simulink model "ECU1119_18b_st"  (R2018b)
settings: Solver=FixedStepDiscrete  StartTime=0.0  StopTime=10.0  RelTol=1e-3
InitFcn:
  | mbd_mpc_consistency_checks(bdroot(gcs));
values from neighbouring files (symbols this model uses):
  ANRtarget = 1.05    [Engine_init.m]
  EGRKi = 0.03    [Engine_init.m]
  EGRKp = 1.2*3    (= 3.6)    [Engine_init.m]
  EGRMax = 1    [Engine_init.m]
  EGRMin = 0    [Engine_init.m]
  EGRTgt = [0.25,0.22,0.20,0.18,0.16,0.12,0.10 ... (first row only)    [Engine_init.m]
  EGRTgt_x = [700,1200,1400,1600,1800,2000,2200]    [Engine_init.m]
  EGRTgt_y = [20,60,100,140,160]    [Engine_init.m]
  EngineSpdTgt = [700:150:2200]    [Engine_init.m]
  EngineSpdTgt_x = [0:10:100]    [Engine_init.m]
  FuelCyleMax = [40,50,60,60,60 ... (first row only)    [Engine_init.m]
  FuelCyleMax_x = [120,180,240,300,360]    [Engine_init.m]
  FuelCyleMax_y = [700,1200,1400,1600,1800,2000,2200]    [Engine_init.m]
  FuelCyleMaxSw = 0    [Engine_init.m]
  FuelCyleMin = 10    [Engine_init.m]
  FuelKd = 0    [Engine_init.m]
  FuelKi = 0.009*5    (= 0.045)    [Engine_init.m]
  FuelKp = 0.03*5    (= 0.15)    [Engine_init.m]
  Regen_Enable_SW = true    [Engine_init.m]
  Soot_Load_Off = 4    [Engine_init.m]
  Soot_Load_On = 18    [Engine_init.m]
  T_regen_max = 680    [Engine_init.m]
  T_regen_min = 550    [Engine_init.m]
undefined symbols (not defined in the file or in its folder): fifo_0_vect, fifo_1_vect, LQFP, pts1_fifo_0_vect, pts1_fifo_1_vect, pts2_fifo_0_vect, pts2_fifo_1_vect, pts3_fifo_0_vect, pts3_fifo_1_vect, pts4_fifo_0_vect, pts4_fifo_1_vect
libraries: mbd_mpc574x_ec_toolbox x111, simulink x12, canmsglib x8
(part 4 of 5)

== system ECU1119_18b_st/SigIn/PWM/PWM_PTS2 ==
  Add : Sum  Inputs=+-  AccumDataTypeStr=single
  Add1 : Sum  Inputs=+-  AccumDataTypeStr=single
  Data Store Memory : DataStoreMemory  DataStoreName=pts2_pwm_cnt  ReadBeforeWriteMsg=warning  WriteAfterWriteMsg=warning  WriteAfterReadMsg=warning  ShowAdditionalParam=off  OutDataTypeStr=uint8
  Data Store Memory2 : DataStoreMemory  DataStoreName=pts2_fifo_1_vect  ReadBeforeWriteMsg=warning  WriteAfterWriteMsg=warning  WriteAfterReadMsg=warning  InitialValue=[0 0 0 0 0 0 0 0]  ShowAdditionalParam=off  OutDataTypeStr=uint16
  Data Store Memory4 : DataStoreMemory  DataStoreName=pts2_fifo_0_vect  ReadBeforeWriteMsg=warning  WriteAfterWriteMsg=warning  WriteAfterReadMsg=warning  InitialValue=[0 0 0 0 0 0 0 0]  ShowAdditionalParam=off  OutDataTypeStr=uint16
  Data Store Read : DataStoreRead  DataStoreName=pts2_fifo_0_vect  DataStoreElements=pts2_fifo_0_vect(2)#pts2_fifo_0_vect(1)
  Data Store Read1 : DataStoreRead  DataStoreName=pts2_fifo_1_vect  DataStoreElements=pts2_fifo_1_vect(1)
  Data Store Read2 : DataStoreRead  DataStoreName=pts2_fifo_0_vect  DataStoreElements=pts2_fifo_0_vect(1)
  Data Store Write3 : DataStoreWrite  DataStoreName=pts2_fifo_0_vect
  Data Store Write5 : DataStoreWrite  DataStoreName=pts2_fifo_1_vect
  Divide : Product  Inputs=*/  OutDataTypeStr=single
  Divide1 : Product  Inputs=*//
  Freq_MC : Constant  Value=80000000  OutDataTypeStr=single
  Prescaler : Constant  Value=32  OutDataTypeStr=single
  Subsystem : Subsystem
  Subsystem_capture : Subsystem
  Terminator1 : Terminator
  Terminator2 : Terminator
  eTimer_ISR : mbd_mpc574x_ec_toolbox/Motor Control Blocks/eTIMER Blocks/eTimer_ISR_Handler  etimerModule=1  etimerInterrupt=Channel Interrupt  etimerChannel=3  etimerIsrPriority=14
      settings: SourceProductName=NXP Model-Based Design Toolbox for MPC57xx MCUs
  DC : Outport
  freq : Outport  Port=2
  wires:
  Subsystem/1(Out1) -> DC/1
  Divide/1 -> Subsystem/1(In1)
  Data Store Read/1 -> Add/1
  Divide1/1 -> freq/1
  Data Store Read2/1 -> Add1/2
  Add1/1 -> Divide/1
  Freq_MC/1 -> Divide1/1
  Data Store Read/2 -> Add/2
  Data Store Read1/1 -> Add1/1
  Add/1 -> Divide1/3, Divide/2
  Prescaler/1 -> Divide1/2
  eTimer_ISR/1 -> Subsystem_capture/Trigger
  Subsystem_capture/2(Out2) -> Data Store Write3/1
  Subsystem_capture/4(Out4) -> Data Store Write5/1
  Subsystem_capture/3(Out3) -> Terminator2/1
  Subsystem_capture/1(Out1) -> Terminator1/1
  eTimer_ISR/2 -> Subsystem_capture/1(In1)

== system ECU1119_18b_st/SigIn/PWM/PWM_PTS3 ==
  Add : Sum  Inputs=+-  AccumDataTypeStr=single
  Add1 : Sum  Inputs=+-  AccumDataTypeStr=single
  Data Store Memory : DataStoreMemory  DataStoreName=pts3_pwm_cnt  ReadBeforeWriteMsg=warning  WriteAfterWriteMsg=warning  WriteAfterReadMsg=warning  ShowAdditionalParam=off  OutDataTypeStr=uint8
  Data Store Memory2 : DataStoreMemory  DataStoreName=pts3_fifo_1_vect  ReadBeforeWriteMsg=warning  WriteAfterWriteMsg=warning  WriteAfterReadMsg=warning  InitialValue=[0 0 0 0 0 0 0 0]  ShowAdditionalParam=off  OutDataTypeStr=uint16
  Data Store Memory4 : DataStoreMemory  DataStoreName=pts3_fifo_0_vect  ReadBeforeWriteMsg=warning  WriteAfterWriteMsg=warning  WriteAfterReadMsg=warning  InitialValue=[0 0 0 0 0 0 0 0]  ShowAdditionalParam=off  OutDataTypeStr=uint16
  Data Store Read : DataStoreRead  DataStoreName=pts3_fifo_0_vect  DataStoreElements=pts3_fifo_0_vect(2)#pts3_fifo_0_vect(1)
  Data Store Read1 : DataStoreRead  DataStoreName=pts3_fifo_1_vect  DataStoreElements=pts3_fifo_1_vect(1)
  Data Store Read2 : DataStoreRead  DataStoreName=pts3_fifo_0_vect  DataStoreElements=pts3_fifo_0_vect(1)
  Data Store Write3 : DataStoreWrite  DataStoreName=pts3_fifo_0_vect
  Data Store Write5 : DataStoreWrite  DataStoreName=pts3_fifo_1_vect
  Divide : Product  Inputs=*/  OutDataTypeStr=single
  Divide1 : Product  Inputs=*//
  Freq_MC : Constant  Value=80000000  OutDataTypeStr=single
  Prescaler : Constant  Value=32  OutDataTypeStr=single
  Subsystem : Subsystem
  Subsystem_capture : Subsystem
  Terminator1 : Terminator
  Terminator2 : Terminator
  eTimer_ISR : mbd_mpc574x_ec_toolbox/Motor Control Blocks/eTIMER Blocks/eTimer_ISR_Handler  etimerModule=1  etimerInterrupt=Channel Interrupt  etimerChannel=1  etimerIsrPriority=14
      settings: SourceProductName=NXP Model-Based Design Toolbox for MPC57xx MCUs
  DC : Outport
  freq : Outport  Port=2
  wires:
  eTimer_ISR/2 -> Subsystem_capture/1(In1)
  Subsystem_capture/1(Out1) -> Terminator1/1
  Subsystem_capture/3(Out3) -> Terminator2/1
  Subsystem_capture/4(Out4) -> Data Store Write5/1
  Subsystem_capture/2(Out2) -> Data Store Write3/1
  eTimer_ISR/1 -> Subsystem_capture/Trigger
  Prescaler/1 -> Divide1/2
  Add/1 -> Divide/2, Divide1/3
  Data Store Read1/1 -> Add1/1
  Data Store Read/2 -> Add/2
  Freq_MC/1 -> Divide1/1
  Add1/1 -> Divide/1
  Data Store Read2/1 -> Add1/2
  Divide1/1 -> freq/1
  Data Store Read/1 -> Add/1
  Divide/1 -> Subsystem/1(In1)
  Subsystem/1(Out1) -> DC/1

== system ECU1119_18b_st/SigIn/PWM/PWM_PTS4 ==
  Add : Sum  Inputs=+-  AccumDataTypeStr=single
  Add1 : Sum  Inputs=+-  AccumDataTypeStr=single
  Data Store Memory : DataStoreMemory  DataStoreName=pts4_pwm_cnt  ReadBeforeWriteMsg=warning  WriteAfterWriteMsg=warning  WriteAfterReadMsg=warning  ShowAdditionalParam=off  OutDataTypeStr=uint8
  Data Store Memory2 : DataStoreMemory  DataStoreName=pts4_fifo_1_vect  ReadBeforeWriteMsg=warning  WriteAfterWriteMsg=warning  WriteAfterReadMsg=warning  InitialValue=[0 0 0 0 0 0 0 0]  ShowAdditionalParam=off  OutDataTypeStr=uint16
  Data Store Memory4 : DataStoreMemory  DataStoreName=pts4_fifo_0_vect  ReadBeforeWriteMsg=warning  WriteAfterWriteMsg=warning  WriteAfterReadMsg=warning  InitialValue=[0 0 0 0 0 0 0 0]  ShowAdditionalParam=off  OutDataTypeStr=uint16
  Data Store Read : DataStoreRead  DataStoreName=pts4_fifo_0_vect  DataStoreElements=pts4_fifo_0_vect(2)#pts4_fifo_0_vect(1)
  Data Store Read1 : DataStoreRead  DataStoreName=pts4_fifo_1_vect  DataStoreElements=pts4_fifo_1_vect(1)
  Data Store Read2 : DataStoreRead  DataStoreName=pts4_fifo_0_vect  DataStoreElements=pts4_fifo_0_vect(1)
  Data Store Write3 : DataStoreWrite  DataStoreName=pts4_fifo_0_vect
  Data Store Write5 : DataStoreWrite  DataStoreName=pts4_fifo_1_vect
  Divide : Product  Inputs=*/  OutDataTypeStr=single
  Divide1 : Product  Inputs=*//
  Freq_MC : Constant  Value=80000000  OutDataTypeStr=single
  Prescaler : Constant  Value=32  OutDataTypeStr=single
  Subsystem : Subsystem
  Subsystem_capture : Subsystem
  Terminator1 : Terminator
  Terminator2 : Terminator
  eTimer_ISR : mbd_mpc574x_ec_toolbox/Motor Control Blocks/eTIMER Blocks/eTimer_ISR_Handler  etimerModule=0  etimerInterrupt=Channel Interrupt  etimerChannel=2  etimerIsrPriority=14
      settings: SourceProductName=NXP Model-Based Design Toolbox for MPC57xx MCUs
  DC : Outport
  freq : Outport  Port=2
  wires:
  Subsystem/1(Out1) -> DC/1
  Divide/1 -> Subsystem/1(In1)
  Data Store Read/1 -> Add/1
  Divide1/1 -> freq/1
  Data Store Read2/1 -> Add1/2
  Add1/1 -> Divide/1
  Freq_MC/1 -> Divide1/1
  Data Store Read/2 -> Add/2
  Data Store Read1/1 -> Add1/1
  Add/1 -> Divide1/3, Divide/2
  Prescaler/1 -> Divide1/2
  eTimer_ISR/1 -> Subsystem_capture/Trigger
  Subsystem_capture/2(Out2) -> Data Store Write3/1
  Subsystem_capture/4(Out4) -> Data Store Write5/1
  Subsystem_capture/3(Out3) -> Terminator2/1
  Subsystem_capture/1(Out1) -> Terminator1/1
  eTimer_ISR/2 -> Subsystem_capture/1(In1)

== system ECU1119_18b_st/SigIn/PWM/Subsystem ==
  Data Store Memory1 : DataStoreMemory  DataStoreName=fifo_1_value  ReadBeforeWriteMsg=warning  WriteAfterWriteMsg=warning  WriteAfterReadMsg=warning  VectorParams1D=off  ShowAdditionalParam=off  OutDataTypeStr=uint16
  Data Store Memory3 : DataStoreMemory  DataStoreName=fifo_0_value  ReadBeforeWriteMsg=warning  WriteAfterWriteMsg=warning  WriteAfterReadMsg=warning  VectorParams1D=off  ShowAdditionalParam=off  OutDataTypeStr=uint16
  Data Store Memory5 : DataStoreMemory  DataStoreName=frequency  ReadBeforeWriteMsg=warning  WriteAfterWriteMsg=warning  WriteAfterReadMsg=warning  VectorParams1D=off  ShowAdditionalParam=off  OutDataTypeStr=single
  Data Store Memory6 : DataStoreMemory  DataStoreName=duty_cycle  ReadBeforeWriteMsg=warning  WriteAfterWriteMsg=warning  WriteAfterReadMsg=warning  VectorParams1D=off  ShowAdditionalParam=off  OutDataTypeStr=single
  Data Store Write10 : DataStoreWrite  DataStoreName=fifo_0_vect
  Data Store Write11 : DataStoreWrite  DataStoreName=fifo_1_value
  Data Store Write12 : DataStoreWrite  DataStoreName=fifo_1_vect
  Data Store Write13 : DataStoreWrite  DataStoreName=duty_cycle
  Data Store Write8 : DataStoreWrite  DataStoreName=frequency
  Data Store Write9 : DataStoreWrite  DataStoreName=fifo_0_value
  Frequency_DutyCycle_Computation : Subsystem
  eTimer Configuration and Signal Measurements : Subsystem
  wires:
  eTimer Configuration and Signal Measurements/4(Out4) -> Data Store Write12/1
  eTimer Configuration and Signal Measurements/2(Out2) -> Data Store Write10/1
  eTimer Configuration and Signal Measurements/3(Out3) -> Data Store Write11/1
  eTimer Configuration and Signal Measurements/1(Out1) -> Data Store Write9/1
  Frequency_DutyCycle_Computation/2(Out2) -> Data Store Write8/1
  Frequency_DutyCycle_Computation/1(Out1) -> Data Store Write13/1

== system ECU1119_18b_st/GPIO /SPI0: LS09_14_15_16_1_2_11_4/LS_CTRL/If Action Subsystem1 ==
  Add : Sum  Inputs=++++
  Constant1 : Constant  Value=128  OutDataTypeStr=uint8
  Constant2 : Constant  Value=64  OutDataTypeStr=uint8
  Constant3 : Constant  Value=32  OutDataTypeStr=uint8
  Constant4 : Constant  Value=16  OutDataTypeStr=uint8
  Constant5 : Constant  Value=8  OutDataTypeStr=uint8
  Constant6 : Constant  Value=4  OutDataTypeStr=uint8
  Constant7 : Constant  Value=2  OutDataTypeStr=uint8
  Constant8 : Constant  OutDataTypeStr=uint8
  Constant9 : Constant  Value=128  OutDataTypeStr=uint8
  Data Store Read : DataStoreRead  DataStoreName=LS004
  Data Store Read4 : DataStoreRead  DataStoreName=LS011
  Data Store Read5 : DataStoreRead  DataStoreName=LS001
  Data Store Read6 : DataStoreRead  DataStoreName=LS002
  Data Type Conversion : DataTypeConversion
  Data Type Conversion1 : DataTypeConversion
  Switch{,1..3} (4 alike) : Switch  Criteria=u2 > Threshold
  Out1 : Outport
  Out2 : Outport  Port=2
  wires:
  Constant2/1 -> Switch/3
  Constant1/1 -> Switch/1
  Add/1 -> Data Type Conversion1/1
  Data Store Read6/1 -> Switch/2
  Constant7/1 -> Switch3/1
  Switch1/1 -> Add/2
  Constant5/1 -> Switch2/1
  Switch/1 -> Add/1
  Constant4/1 -> Switch1/3
  Data Store Read/1 -> Switch3/2
  Switch2/1 -> Add/3
  Data Store Read4/1 -> Switch2/2
  Switch3/1 -> Add/4
  Constant3/1 -> Switch1/1
  Data Store Read5/1 -> Switch1/2
  Constant8/1 -> Switch3/3
  Constant9/1 -> Data Type Conversion/1
  Constant6/1 -> Switch2/3
  Data Type Conversion/1 -> Out1/1
  Data Type Conversion1/1 -> Out2/1

== system ECU1119_18b_st/GPIO /SPI0: LS09_14_15_16_1_2_11_4/LS_CTRL1/If Action Subsystem1 ==
  Add : Sum  Inputs=++++
  Constant1 : Constant  Value=128  OutDataTypeStr=uint8
  Constant2 : Constant  Value=64  OutDataTypeStr=uint8
  Constant3 : Constant  Value=32  OutDataTypeStr=uint8
  Constant4 : Constant  Value=16  OutDataTypeStr=uint8
  Constant5 : Constant  Value=8  OutDataTypeStr=uint8
  Constant6 : Constant  Value=4  OutDataTypeStr=uint8
  Constant7 : Constant  Value=2  OutDataTypeStr=uint8
  Constant8 : Constant  OutDataTypeStr=uint8
  Constant9 : Constant  Value=128  OutDataTypeStr=uint8
  Data Store Read : DataStoreRead  DataStoreName=LS014
  Data Store Read4 : DataStoreRead  DataStoreName=LS015
  Data Store Read5 : DataStoreRead  DataStoreName=LS009
  Data Store Read6 : DataStoreRead  DataStoreName=LS016
  Data Type Conversion : DataTypeConversion
  Data Type Conversion1 : DataTypeConversion
  Switch{,1..3} (4 alike) : Switch  Criteria=u2 > Threshold
  Out1 : Outport
  Out2 : Outport  Port=2
  wires:
  Data Type Conversion1/1 -> Out2/1
  Data Type Conversion/1 -> Out1/1
  Constant6/1 -> Switch2/3
  Constant9/1 -> Data Type Conversion/1
  Constant8/1 -> Switch3/3
  Data Store Read5/1 -> Switch1/2
  Constant3/1 -> Switch1/1
  Switch3/1 -> Add/4
  Data Store Read4/1 -> Switch2/2
  Switch2/1 -> Add/3
  Data Store Read/1 -> Switch3/2
  Constant4/1 -> Switch1/3
  Switch/1 -> Add/1
  Constant5/1 -> Switch2/1
  Switch1/1 -> Add/2
  Constant7/1 -> Switch3/1
  Data Store Read6/1 -> Switch/2
  Add/1 -> Data Type Conversion1/1
  Constant1/1 -> Switch/1
  Constant2/1 -> Switch/3

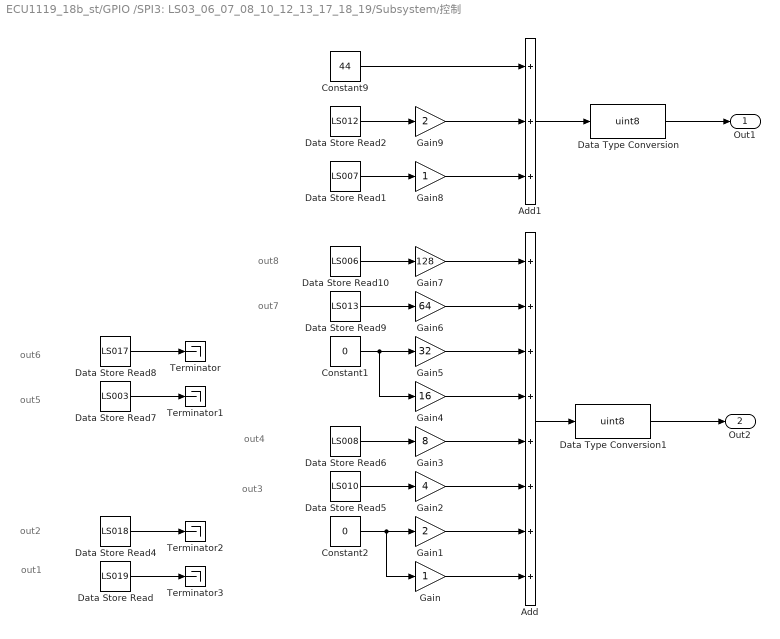
== system ECU1119_18b_st/GPIO /SPI3: LS03_06_07_08_10_12_13_17_18_19/Subsystem/控制 ==
  note: out1
  note: out2
  note: out3
  note: out5
  note: out4
  note: out7
  note: out6
  note: out8
  Add : Sum  Inputs=++++++++
  Add1 : Sum  Inputs=+++
  Constant1 : Constant  Value=0
  Constant2 : Constant  Value=0
  Constant9 : Constant  Value=44  OutDataTypeStr=uint8
  Data Store Read : DataStoreRead  DataStoreName=LS019
  Data Store Read1 : DataStoreRead  DataStoreName=LS007
  Data Store Read10 : DataStoreRead  DataStoreName=LS006
  Data Store Read2 : DataStoreRead  DataStoreName=LS012
  Data Store Read4 : DataStoreRead  DataStoreName=LS018
  Data Store Read5 : DataStoreRead  DataStoreName=LS010
  Data Store Read6 : DataStoreRead  DataStoreName=LS008
  Data Store Read7 : DataStoreRead  DataStoreName=LS003
  Data Store Read8 : DataStoreRead  DataStoreName=LS017
  Data Store Read9 : DataStoreRead  DataStoreName=LS013
  Data Type Conversion : DataTypeConversion  OutDataTypeStr=uint8
  Data Type Conversion1 : DataTypeConversion  OutDataTypeStr=uint8
  Gain : Gain
  Gain1 : Gain  Gain=2
  Gain2 : Gain  Gain=4
  Gain3 : Gain  Gain=8
  Gain4 : Gain  Gain=16
  Gain5 : Gain  Gain=32
  Gain6 : Gain  Gain=64
  Gain7 : Gain  Gain=128
  Gain8 : Gain
  Gain9 : Gain  Gain=2
  Terminator{,1..3} (4 alike) : Terminator
  Out1 : Outport  VectorParamsAs1DForOutWhenUnconnected=on
  Out2 : Outport  Port=2  VectorParamsAs1DForOutWhenUnconnected=on
  wires:
  Constant9/1 -> Add1/1
  Data Store Read10/1 -> Gain7/1
  Data Type Conversion1/1 -> Out2/1
  Data Store Read2/1 -> Gain9/1
  Add1/1 -> Data Type Conversion/1
  Add/1 -> Data Type Conversion1/1
  Data Store Read5/1 -> Gain2/1
  Gain6/1 -> Add/2
  Data Store Read1/1 -> Gain8/1
  Gain9/1 -> Add1/2
  Gain7/1 -> Add/1
  Gain/1 -> Add/8
  Data Type Conversion/1 -> Out1/1
  Data Store Read9/1 -> Gain6/1
  Gain4/1 -> Add/4
  Gain8/1 -> Add1/3
  Gain1/1 -> Add/7
  Data Store Read6/1 -> Gain3/1
  Gain3/1 -> Add/5
  Gain2/1 -> Add/6
  Gain5/1 -> Add/3
  Data Store Read8/1 -> Terminator/1
  Data Store Read7/1 -> Terminator1/1
  Constant1/1 -> Gain4/1, Gain5/1
  Data Store Read/1 -> Terminator3/1
  Data Store Read4/1 -> Terminator2/1
  Constant2/1 -> Gain/1, Gain1/1

== system ECU1119_18b_st/Initialization & SPI timer1/CS1 LS/Subsystem/SPI_en ==
  Action Port : ActionPort
  Add : Sum
  Add1 : Sum  Inputs=+++
  Constant1 : Constant  Value=0
  Constant11 : Constant  OutDataTypeStr=uint8
  Constant2 : Constant  OutDataTypeStr=uint8
  Constant3 : Constant  Value=0
  Constant9 : Constant  Value=128  OutDataTypeStr=uint8
  Data Type Conversion : DataTypeConversion
  Data Type Conversion1 : DataTypeConversion
  Gain : Gain  Gain=64
  Out1 : Outport
  Out2 : Outport  Port=2
  wires:
  Constant1/1 -> Add/1
  Constant9/1 -> Add1/1
  Add1/1 -> Data Type Conversion/1
  Constant11/1 -> Add1/2
  Constant2/1 -> Gain/1
  Gain/1 -> Add1/3
  Add/1 -> Data Type Conversion1/1
  Constant3/1 -> Add/2
  Data Type Conversion/1 -> Out1/1
  Data Type Conversion1/1 -> Out2/1

== system ECU1119_18b_st/Initialization & SPI timer1/CS1 LS/Subsystem/clear  ==
  Action Port : ActionPort
  Add : Sum
  Add1 : Sum  Inputs=+++
  Constant1 : Constant
  Constant11 : Constant  Value=7  OutDataTypeStr=uint8
  Constant2 : Constant  Value=0  OutDataTypeStr=uint8
  Constant3 : Constant  Value=0
  Constant9 : Constant  Value=128  OutDataTypeStr=uint8
  Data Type Conversion : DataTypeConversion
  Data Type Conversion1 : DataTypeConversion
  Gain : Gain  Gain=64
  Out1 : Outport
  Out2 : Outport  Port=2
  wires:
  Constant3/1 -> Add/2
  Add/1 -> Data Type Conversion1/1
  Gain/1 -> Add1/3
  Constant2/1 -> Gain/1
  Constant11/1 -> Add1/2
  Add1/1 -> Data Type Conversion/1
  Data Type Conversion1/1 -> Out2/1
  Data Type Conversion/1 -> Out1/1
  Constant9/1 -> Add1/1
  Constant1/1 -> Add/1

== system ECU1119_18b_st/Initialization & SPI timer1/CS1 LS/Subsystem/confi_enbit ==
  Action Port : ActionPort
  Add : Sum
  Add1 : Sum  Inputs=+++
  Constant1 : Constant
  Constant11 : Constant  Value=7  OutDataTypeStr=uint8
  Constant2 : Constant  OutDataTypeStr=uint8
  Constant3 : Constant  Value=128
  Constant9 : Constant  Value=128  OutDataTypeStr=uint8
  Data Type Conversion : DataTypeConversion
  Data Type Conversion1 : DataTypeConversion
  Gain : Gain  Gain=64
  Out1 : Outport
  Out2 : Outport  Port=2
  wires:
  Constant1/1 -> Add/1
  Constant9/1 -> Add1/1
  Add1/1 -> Data Type Conversion/1
  Constant11/1 -> Add1/2
  Constant2/1 -> Gain/1
  Gain/1 -> Add1/3
  Add/1 -> Data Type Conversion1/1
  Constant3/1 -> Add/2
  Data Type Conversion/1 -> Out1/1
  Data Type Conversion1/1 -> Out2/1

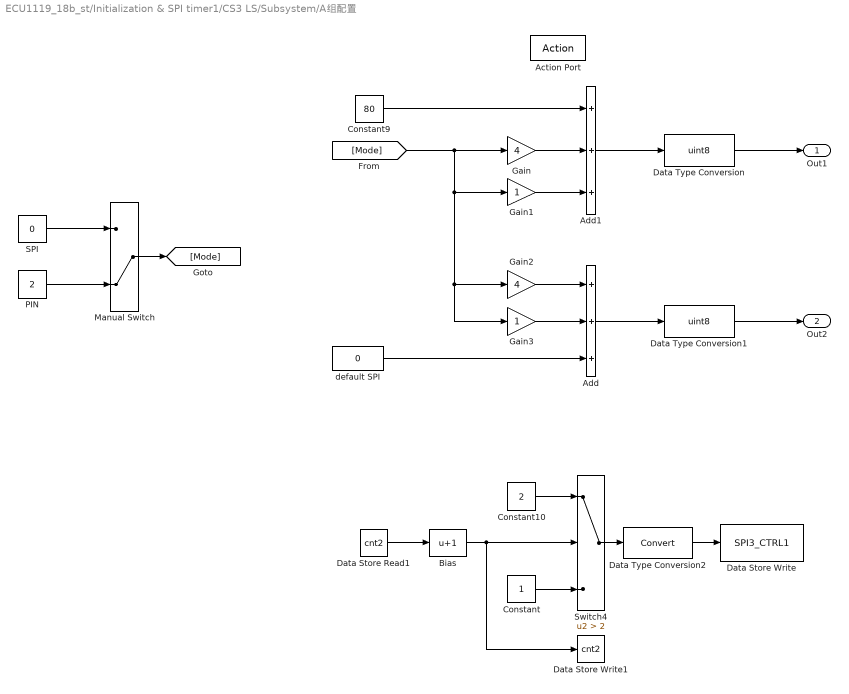
== system ECU1119_18b_st/Initialization & SPI timer1/CS3 LS/Subsystem/A组配置 ==
  Action Port : ActionPort
  Add : Sum  Inputs=+++
  Add1 : Sum  Inputs=+++
  Bias : Bias  Bias=1
  Constant : Constant
  Constant10 : Constant  Value=2
  Constant9 : Constant  Value=80  OutDataTypeStr=uint8
  Data Store Read1 : DataStoreRead  DataStoreName=cnt2
  Data Store Write : DataStoreWrite  DataStoreName=SPI3_CTRL1
  Data Store Write1 : DataStoreWrite  DataStoreName=cnt2
  Data Type Conversion : DataTypeConversion  OutDataTypeStr=uint8
  Data Type Conversion1 : DataTypeConversion  OutDataTypeStr=uint8
  Data Type Conversion2 : DataTypeConversion
  Gain : Gain  Gain=4
  Gain1 : Gain
  Gain2 : Gain  Gain=4
  Gain3 : Gain
  Manual Switch : ManualSwitch  CurrentSetting=0
  PIN : Constant  Value=2
  SPI : Constant  Value=0
  Switch4 : Switch  Criteria=u2 > Threshold  Threshold=2
  default SPI : Constant  Value=0
  Out1 : Outport  VectorParamsAs1DForOutWhenUnconnected=on
  Out2 : Outport  Port=2  VectorParamsAs1DForOutWhenUnconnected=on
  wires:
  Switch4/1 -> Data Type Conversion2/1
  Constant/1 -> Switch4/3
  Constant10/1 -> Switch4/1
  Data Store Read1/1 -> Bias/1
  Bias/1 -> Data Store Write1/1, Switch4/2
  Data Type Conversion2/1 -> Data Store Write/1
  Data Type Conversion/1 -> Out1/1
  Data Type Conversion1/1 -> Out2/1
  Constant9/1 -> Add1/1
  Add/1 -> Data Type Conversion1/1
  [Mode] -> Gain3/1, Gain2/1, Gain1/1, Gain/1
  Gain2/1 -> Add/1
  Gain3/1 -> Add/2
  default SPI/1 -> Add/3
  Add1/1 -> Data Type Conversion/1
  Gain/1 -> Add1/2
  Gain1/1 -> Add1/3
  SPI/1 -> Manual Switch/1
  Manual Switch/1 -> [Mode]
  PIN/1 -> Manual Switch/2

== system ECU1119_18b_st/Initialization & SPI timer1/CS3 LS/Subsystem/B组配置 ==
  Action Port : ActionPort
  Bias : Bias  Bias=1
  Constant : Constant  Value=2
  Constant1 : Constant  Value=0  OutDataTypeStr=uint8
  Constant10 : Constant  Value=3
  Constant9 : Constant  Value=96  OutDataTypeStr=uint8
  Data Store Read1 : DataStoreRead  DataStoreName=cnt2
  Data Store Write : DataStoreWrite  DataStoreName=SPI3_CTRL1
  Data Store Write1 : DataStoreWrite  DataStoreName=cnt2
  Data Type Conversion : DataTypeConversion  OutDataTypeStr=uint8
  Data Type Conversion1 : DataTypeConversion  OutDataTypeStr=uint8
  Data Type Conversion2 : DataTypeConversion
  Switch4 : Switch  Criteria=u2 > Threshold  Threshold=4
  Out1 : Outport  VectorParamsAs1DForOutWhenUnconnected=on
  Out2 : Outport  Port=2  VectorParamsAs1DForOutWhenUnconnected=on
  wires:
  Data Type Conversion2/1 -> Data Store Write/1
  Bias/1 -> Switch4/2, Data Store Write1/1
  Data Store Read1/1 -> Bias/1
  Constant10/1 -> Switch4/1
  Constant/1 -> Switch4/3
  Switch4/1 -> Data Type Conversion2/1
  Constant1/1 -> Data Type Conversion1/1
  Data Type Conversion/1 -> Out1/1
  Constant9/1 -> Data Type Conversion/1
  Data Type Conversion1/1 -> Out2/1

== system ECU1119_18b_st/Initialization & SPI timer1/CS5 LS/Subsystem/SPI_en ==
  Action Port : ActionPort
  Add : Sum
  Add1 : Sum  Inputs=+++
  Constant1 : Constant  Value=0
  Constant11 : Constant  OutDataTypeStr=uint8
  Constant2 : Constant  OutDataTypeStr=uint8
  Constant3 : Constant  Value=0
  Constant9 : Constant  Value=128  OutDataTypeStr=uint8
  Data Type Conversion : DataTypeConversion
  Data Type Conversion1 : DataTypeConversion
  Gain : Gain  Gain=64
  Out1 : Outport
  Out2 : Outport  Port=2
  wires:
  Constant1/1 -> Add/1
  Constant9/1 -> Add1/1
  Add1/1 -> Data Type Conversion/1
  Constant11/1 -> Add1/2
  Constant2/1 -> Gain/1
  Gain/1 -> Add1/3
  Add/1 -> Data Type Conversion1/1
  Constant3/1 -> Add/2
  Data Type Conversion/1 -> Out1/1
  Data Type Conversion1/1 -> Out2/1

== system ECU1119_18b_st/Initialization & SPI timer1/CS5 LS/Subsystem/clear  ==
  Action Port : ActionPort
  Add : Sum
  Add1 : Sum  Inputs=+++
  Constant1 : Constant
  Constant11 : Constant  Value=7  OutDataTypeStr=uint8
  Constant2 : Constant  Value=0  OutDataTypeStr=uint8
  Constant3 : Constant  Value=0
  Constant9 : Constant  Value=128  OutDataTypeStr=uint8
  Data Type Conversion : DataTypeConversion
  Data Type Conversion1 : DataTypeConversion
  Gain : Gain  Gain=64
  Out1 : Outport
  Out2 : Outport  Port=2
  wires:
  Constant3/1 -> Add/2
  Add/1 -> Data Type Conversion1/1
  Gain/1 -> Add1/3
  Constant2/1 -> Gain/1
  Constant11/1 -> Add1/2
  Add1/1 -> Data Type Conversion/1
  Data Type Conversion1/1 -> Out2/1
  Data Type Conversion/1 -> Out1/1
  Constant9/1 -> Add1/1
  Constant1/1 -> Add/1

== system ECU1119_18b_st/Initialization & SPI timer1/CS5 LS/Subsystem/confi_enbit ==
  Action Port : ActionPort
  Add : Sum
  Add1 : Sum  Inputs=+++
  Constant1 : Constant
  Constant11 : Constant  Value=7  OutDataTypeStr=uint8
  Constant2 : Constant  OutDataTypeStr=uint8
  Constant3 : Constant  Value=128
  Constant9 : Constant  Value=128  OutDataTypeStr=uint8
  Data Type Conversion : DataTypeConversion
  Data Type Conversion1 : DataTypeConversion
  Gain : Gain  Gain=64
  Out1 : Outport
  Out2 : Outport  Port=2
  wires:
  Constant1/1 -> Add/1
  Constant9/1 -> Add1/1
  Add1/1 -> Data Type Conversion/1
  Constant11/1 -> Add1/2
  Constant2/1 -> Gain/1
  Gain/1 -> Add1/3
  Add/1 -> Data Type Conversion1/1
  Constant3/1 -> Add/2
  Data Type Conversion/1 -> Out1/1
  Data Type Conversion1/1 -> Out2/1

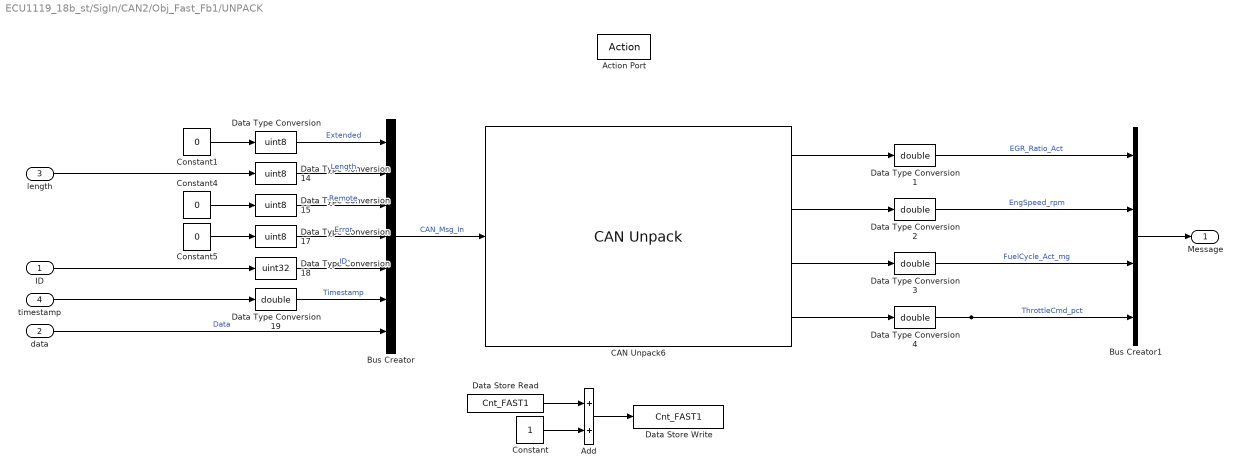
== system ECU1119_18b_st/SigIn/CAN2/Obj_Fast_Fb1/UNPACK ==
  ID : Inport
  data : Inport  Port=2
  length : Inport  Port=3
  timestamp : Inport  Port=4
  Action Port : ActionPort  ActionType=case
  Add : Sum
  Bus Creator : BusCreator  Inputs=7  OutDataTypeStr=Bus: CAN_MESSAGE_BUS  NonVirtualBus=on
  Bus Creator1 : BusCreator  Inputs=4
  CAN Unpack6 : canmsglib/CAN Unpack  CANdbFile=D:\VCU\VCU_Tractor_HaerBin\Tractor2\CANtest\ECU_CAN_st.dbc  MsgList=Obj_Fast_Fb1  MsgName=Obj_Fast_Fb1  MsgIDType=Standard (11-bit identifier)  MsgIdentifier=257  MsgLength=8  SignalInfo=EGR_Ratio_Act$32$16$1$2$1$0$1.000000e-03$0$0$50$#EngSpeed_rpm$0$16$1$2$1$0$1.000000e-01$0$0$3000$#FuelCycle_Act_mg$16$16$1$2$1$0$5.000000e-03$0$0$200$#ThrottleCmd_pct$48$16$1$2$1$0$1.000000e-02$0$0$100$#  NSignals=4  IDPort=off  TimestampPort=off  ErrorPort=off  RemotePort=off  LengthPort=off  StatusPort=off  StartBits=str2num('[int32(32);int32(0);int32(16);int32(48)]')  SignalSizes=str2num('[int32(16);int32(16);int32(16);int32(16)]')  ByteOrders=str2num('[int32(1);int32(1);int32(1);int32(1)]')  DataTypes=str2num('[int32(2);int32(2);int32(2);int32(2)]')  MultiplexTypes=str2num('[int32(1);int32(1);int32(1);int32(1)]')  MultiplexValues=str2num('[double(0);double(0);double(0);double(0)]')  Factors=str2num('[double(1.000000e-03);double(1.000000e-01);double(5.000000e-03);double(1.000000e-02)]')  Offsets=str2num('[double(0);double(0);double(0);double(0)]')  Minimums=str2num('[double(0);double(0);double(0);double(0)]')  Maximums=str2num('[double(50);double(3000);double(200);double(100)]')  ApplyMinMax=off
      settings: SourceProductName=Simulink Real-Time  SourceProductBaseCode=XP  DataFormat=CANdb specified signals
  Constant : Constant  OutDataTypeStr=uint8
  Constant1 : Constant  Value=0  OutDataTypeStr=uint8
  Constant4 : Constant  Value=0  OutDataTypeStr=uint8
  Constant5 : Constant  Value=0  OutDataTypeStr=uint8
  Data Store Read : DataStoreRead  DataStoreName=Cnt_FAST1
  Data Store Write : DataStoreWrite  DataStoreName=Cnt_FAST1
  Data Type Conversion{,14..15,17} (4 alike) : DataTypeConversion  OutDataTypeStr=uint8
  Data Type Conversion{1..4,19} (5 alike) : DataTypeConversion  OutDataTypeStr=double
  Data Type Conversion18 : DataTypeConversion  OutDataTypeStr=uint32
  Message : Outport
  wires:
  Bus Creator1/1 -> Message/1
  Data Type Conversion15/1 -> Bus Creator/3  "Remote"
  Data Type Conversion14/1 -> Bus Creator/2  "Length"
  Data Type Conversion/1 -> Bus Creator/1  "Extended"
  Bus Creator/1 -> CAN Unpack6/1  "CAN_Msg_In"
  Data Type Conversion17/1 -> Bus Creator/4  "Error"
  timestamp/1 -> Data Type Conversion19/1
  Data Type Conversion19/1 -> Bus Creator/6  "Timestamp"
  ID/1 -> Data Type Conversion18/1
  Constant5/1 -> Data Type Conversion17/1
  Constant1/1 -> Data Type Conversion/1
  Data Type Conversion18/1 -> Bus Creator/5  "ID"
  data/1 -> Bus Creator/7  "Data"
  length/1 -> Data Type Conversion14/1
  Constant4/1 -> Data Type Conversion15/1
  CAN Unpack6/1 -> Data Type Conversion1/1
  CAN Unpack6/2 -> Data Type Conversion2/1
  CAN Unpack6/3 -> Data Type Conversion3/1
  CAN Unpack6/4 -> Data Type Conversion4/1
  Data Type Conversion1/1 -> Bus Creator1/1  "EGR_Ratio_Act"
  Data Type Conversion2/1 -> Bus Creator1/2  "EngSpeed_rpm"
  Data Type Conversion3/1 -> Bus Creator1/3  "FuelCycle_Act_mg"
  Data Type Conversion4/1 -> Bus Creator1/4  "ThrottleCmd_pct"
  Add/1 -> Data Store Write/1
  Constant/1 -> Add/2
  Data Store Read/1 -> Add/1

== system ECU1119_18b_st/SigIn/CAN2/Obj_Fast_Fb2/UNPACK ==
  ID : Inport
  data : Inport  Port=2
  length : Inport  Port=3
  timestamp : Inport  Port=4
  Action Port : ActionPort  ActionType=case
  Add : Sum
  Bus Creator : BusCreator  Inputs=7  OutDataTypeStr=Bus: CAN_MESSAGE_BUS  NonVirtualBus=on
  Bus Creator1 : BusCreator  Inputs=3
  CAN Unpack6 : canmsglib/CAN Unpack  CANdbFile=D:\VCU\VCU_Tractor_HaerBin\Tractor2\CANtest\ECU_CAN_st.dbc  MsgList=Obj_Fast_Fb2  MsgName=Obj_Fast_Fb2  MsgIDType=Standard (11-bit identifier)  MsgIdentifier=258  MsgLength=8  SignalInfo=IntakeMass_kgph$16$16$1$2$1$0$1.000000e-01$0$0$1500$#RailPrs_kpa$0$16$1$2$1$0$5$0$0$2000$#Reserved_0300$32$32$1$2$1$0$1$0$0$4294967295$#  NSignals=3  IDPort=off  TimestampPort=off  ErrorPort=off  RemotePort=off  LengthPort=off  StatusPort=off  StartBits=str2num('[int32(16);int32(0);int32(32)]')  SignalSizes=str2num('[int32(16);int32(16);int32(32)]')  ByteOrders=str2num('[int32(1);int32(1);int32(1)]')  DataTypes=str2num('[int32(2);int32(2);int32(2)]')  MultiplexTypes=str2num('[int32(1);int32(1);int32(1)]')  MultiplexValues=str2num('[double(0);double(0);double(0)]')  Factors=str2num('[double(1.000000e-01);double(5);double(1)]')  Offsets=str2num('[double(0);double(0);double(0)]')  Minimums=str2num('[double(0);double(0);double(0)]')  Maximums=str2num('[double(1500);double(2000);double(4294967295)]')  ApplyMinMax=off
      settings: SourceProductName=Simulink Real-Time  SourceProductBaseCode=XP  DataFormat=CANdb specified signals
  Constant : Constant  OutDataTypeStr=uint8
  Constant1 : Constant  Value=0  OutDataTypeStr=uint8
  Constant4 : Constant  Value=0  OutDataTypeStr=uint8
  Constant5 : Constant  Value=0  OutDataTypeStr=uint8
  Data Store Read : DataStoreRead  DataStoreName=Cnt_FAST2
  Data Store Write : DataStoreWrite  DataStoreName=Cnt_FAST2
  Data Type Conversion{,14..15,17} (4 alike) : DataTypeConversion  OutDataTypeStr=uint8
  Data Type Conversion{1..2,4,19} (4 alike) : DataTypeConversion  OutDataTypeStr=double
  Data Type Conversion18 : DataTypeConversion  OutDataTypeStr=uint32
  Message : Outport
  wires:
  Data Store Read/1 -> Add/1
  Constant/1 -> Add/2
  Add/1 -> Data Store Write/1
  Data Type Conversion2/1 -> Bus Creator1/3  "Reserved_0300"
  Data Type Conversion1/1 -> Bus Creator1/2  "RailPrs_kpa"
  Data Type Conversion4/1 -> Bus Creator1/1  "IntakeMass_kgph"
  CAN Unpack6/3 -> Data Type Conversion2/1
  CAN Unpack6/2 -> Data Type Conversion1/1
  CAN Unpack6/1 -> Data Type Conversion4/1
  Constant4/1 -> Data Type Conversion15/1
  length/1 -> Data Type Conversion14/1
  data/1 -> Bus Creator/7  "Data"
  Data Type Conversion18/1 -> Bus Creator/5  "ID"
  Constant1/1 -> Data Type Conversion/1
  Constant5/1 -> Data Type Conversion17/1
  ID/1 -> Data Type Conversion18/1
  Data Type Conversion19/1 -> Bus Creator/6  "Timestamp"
  timestamp/1 -> Data Type Conversion19/1
  Data Type Conversion17/1 -> Bus Creator/4  "Error"
  Bus Creator/1 -> CAN Unpack6/1  "CAN_Msg_In"
  Data Type Conversion/1 -> Bus Creator/1  "Extended"
  Data Type Conversion14/1 -> Bus Creator/2  "Length"
  Data Type Conversion15/1 -> Bus Creator/3  "Remote"
  Bus Creator1/1 -> Message/1

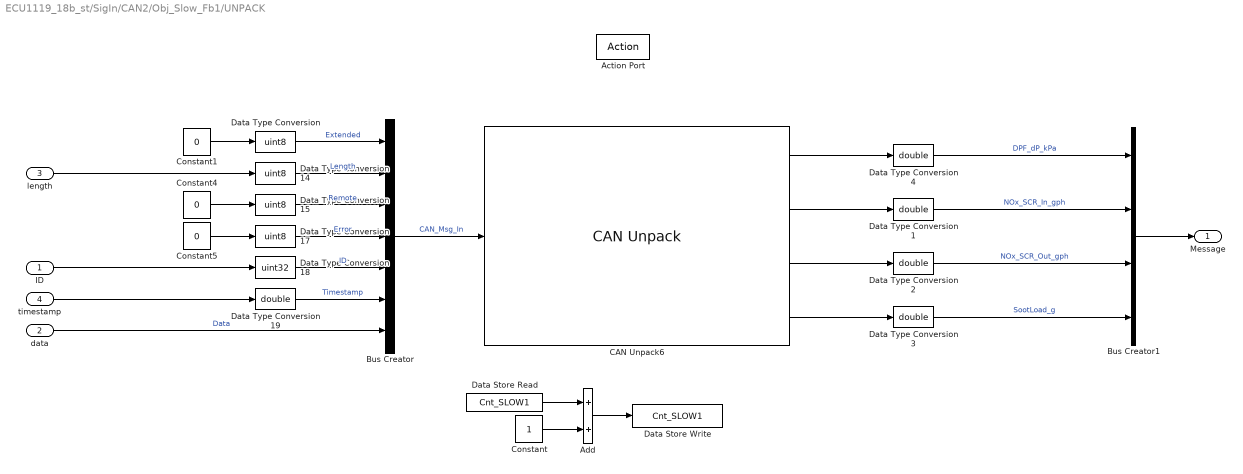
== system ECU1119_18b_st/SigIn/CAN2/Obj_Slow_Fb1/UNPACK ==
  ID : Inport
  data : Inport  Port=2
  length : Inport  Port=3
  timestamp : Inport  Port=4
  Action Port : ActionPort  ActionType=case
  Add : Sum
  Bus Creator : BusCreator  Inputs=7  OutDataTypeStr=Bus: CAN_MESSAGE_BUS  NonVirtualBus=on
  Bus Creator1 : BusCreator  Inputs=4
  CAN Unpack6 : canmsglib/CAN Unpack  CANdbFile=D:\VCU\VCU_Tractor_HaerBin\Tractor2\CANtest\ECU_CAN_st.dbc  MsgList=Obj_Slow_Fb1  MsgName=Obj_Slow_Fb1  MsgIDType=Standard (11-bit identifier)  MsgIdentifier=261  MsgLength=8  SignalInfo=DPF_dP_kPa$16$16$1$2$1$0$1.000000e-02$0$0$20$#NOx_SCR_In_gph$32$16$1$2$1$0$1.000000e-01$0$0$2000$#NOx_SCR_Out_gph$48$16$1$2$1$0$1.000000e-01$0$0$2000$#SootLoad_g$0$16$1$2$1$0$1.000000e-02$0$0$80$#  NSignals=4  IDPort=off  TimestampPort=off  ErrorPort=off  RemotePort=off  LengthPort=off  StatusPort=off  StartBits=str2num('[int32(16);int32(32);int32(48);int32(0)]')  SignalSizes=str2num('[int32(16);int32(16);int32(16);int32(16)]')  ByteOrders=str2num('[int32(1);int32(1);int32(1);int32(1)]')  DataTypes=str2num('[int32(2);int32(2);int32(2);int32(2)]')  MultiplexTypes=str2num('[int32(1);int32(1);int32(1);int32(1)]')  MultiplexValues=str2num('[double(0);double(0);double(0);double(0)]')  Factors=str2num('[double(1.000000e-02);double(1.000000e-01);double(1.000000e-01);double(1.000000e-02)]')  Offsets=str2num('[double(0);double(0);double(0);double(0)]')  Minimums=str2num('[double(0);double(0);double(0);double(0)]')  Maximums=str2num('[double(20);double(2000);double(2000);double(80)]')  ApplyMinMax=off
      settings: SourceProductName=Simulink Real-Time  SourceProductBaseCode=XP  DataFormat=CANdb specified signals
  Constant : Constant  OutDataTypeStr=uint8
  Constant1 : Constant  Value=0  OutDataTypeStr=uint8
  Constant4 : Constant  Value=0  OutDataTypeStr=uint8
  Constant5 : Constant  Value=0  OutDataTypeStr=uint8
  Data Store Read : DataStoreRead  DataStoreName=Cnt_SLOW1
  Data Store Write : DataStoreWrite  DataStoreName=Cnt_SLOW1
  Data Type Conversion{,14..15,17} (4 alike) : DataTypeConversion  OutDataTypeStr=uint8
  Data Type Conversion{1..4,19} (5 alike) : DataTypeConversion  OutDataTypeStr=double
  Data Type Conversion18 : DataTypeConversion  OutDataTypeStr=uint32
  Message : Outport
  wires:
  CAN Unpack6/4 -> Data Type Conversion3/1
  Data Type Conversion3/1 -> Bus Creator1/4  "SootLoad_g"
  Data Store Read/1 -> Add/1
  Constant/1 -> Add/2
  Add/1 -> Data Store Write/1
  Data Type Conversion2/1 -> Bus Creator1/3  "NOx_SCR_Out_gph"
  Data Type Conversion1/1 -> Bus Creator1/2  "NOx_SCR_In_gph"
  Data Type Conversion4/1 -> Bus Creator1/1  "DPF_dP_kPa"
  CAN Unpack6/3 -> Data Type Conversion2/1
  CAN Unpack6/2 -> Data Type Conversion1/1
  CAN Unpack6/1 -> Data Type Conversion4/1
  Constant4/1 -> Data Type Conversion15/1
  length/1 -> Data Type Conversion14/1
  data/1 -> Bus Creator/7  "Data"
  Data Type Conversion18/1 -> Bus Creator/5  "ID"
  Constant1/1 -> Data Type Conversion/1
  Constant5/1 -> Data Type Conversion17/1
  ID/1 -> Data Type Conversion18/1
  Data Type Conversion19/1 -> Bus Creator/6  "Timestamp"
  timestamp/1 -> Data Type Conversion19/1
  Data Type Conversion17/1 -> Bus Creator/4  "Error"
  Bus Creator/1 -> CAN Unpack6/1  "CAN_Msg_In"
  Data Type Conversion/1 -> Bus Creator/1  "Extended"
  Data Type Conversion14/1 -> Bus Creator/2  "Length"
  Data Type Conversion15/1 -> Bus Creator/3  "Remote"
  Bus Creator1/1 -> Message/1

== system ECU1119_18b_st/SigIn/CAN2/Obj_Slow_Fb2/UNPACK ==
  ID : Inport
  data : Inport  Port=2
  length : Inport  Port=3
  timestamp : Inport  Port=4
  Action Port : ActionPort  ActionType=case
  Add : Sum
  Bus Creator : BusCreator  Inputs=7  OutDataTypeStr=Bus: CAN_MESSAGE_BUS  NonVirtualBus=on
  Bus Creator1 : BusCreator  Inputs=4
  CAN Unpack6 : canmsglib/CAN Unpack  CANdbFile=D:\VCU\VCU_Tractor_HaerBin\Tractor2\CANtest\ECU_CAN_st.dbc  MsgList=Obj_Slow_Fb2  MsgName=Obj_Slow_Fb2  MsgIDType=Standard (11-bit identifier)  MsgIdentifier=262  MsgLength=8  SignalInfo=NH3_Store_g$0$16$1$2$1$0$1.000000e-02$0$0$10$#O2_frac_pct$16$16$1$2$1$0$1.000000e-02$0$0$21$#Regen_State$32$4$1$2$1$0$1$0$0$15$#Reserved_0700$36$28$1$2$1$0$1$0$0$268435455$#  NSignals=4  IDPort=off  TimestampPort=off  ErrorPort=off  RemotePort=off  LengthPort=off  StatusPort=off  StartBits=str2num('[int32(0);int32(16);int32(32);int32(36)]')  SignalSizes=str2num('[int32(16);int32(16);int32(4);int32(28)]')  ByteOrders=str2num('[int32(1);int32(1);int32(1);int32(1)]')  DataTypes=str2num('[int32(2);int32(2);int32(2);int32(2)]')  MultiplexTypes=str2num('[int32(1);int32(1);int32(1);int32(1)]')  MultiplexValues=str2num('[double(0);double(0);double(0);double(0)]')  Factors=str2num('[double(1.000000e-02);double(1.000000e-02);double(1);double(1)]')  Offsets=str2num('[double(0);double(0);double(0);double(0)]')  Minimums=str2num('[double(0);double(0);double(0);double(0)]')  Maximums=str2num('[double(10);double(21);double(15);double(268435455)]')  ApplyMinMax=off
      settings: SourceProductName=Simulink Real-Time  SourceProductBaseCode=XP  DataFormat=CANdb specified signals
  Constant : Constant  OutDataTypeStr=uint8
  Constant1 : Constant  Value=0  OutDataTypeStr=uint8
  Constant4 : Constant  Value=0  OutDataTypeStr=uint8
  Constant5 : Constant  Value=0  OutDataTypeStr=uint8
  Data Store Read : DataStoreRead  DataStoreName=Cnt_SLOW2
  Data Store Write : DataStoreWrite  DataStoreName=Cnt_SLOW2
  Data Type Conversion{,14..15,17} (4 alike) : DataTypeConversion  OutDataTypeStr=uint8
  Data Type Conversion{1..4,19} (5 alike) : DataTypeConversion  OutDataTypeStr=double
  Data Type Conversion18 : DataTypeConversion  OutDataTypeStr=uint32
  Message : Outport
  wires:
  Bus Creator1/1 -> Message/1
  Data Type Conversion15/1 -> Bus Creator/3  "Remote"
  Data Type Conversion14/1 -> Bus Creator/2  "Length"
  Data Type Conversion/1 -> Bus Creator/1  "Extended"
  Bus Creator/1 -> CAN Unpack6/1  "CAN_Msg_In"
  Data Type Conversion17/1 -> Bus Creator/4  "Error"
  timestamp/1 -> Data Type Conversion19/1
  Data Type Conversion19/1 -> Bus Creator/6  "Timestamp"
  ID/1 -> Data Type Conversion18/1
  Constant5/1 -> Data Type Conversion17/1
  Constant1/1 -> Data Type Conversion/1
  Data Type Conversion18/1 -> Bus Creator/5  "ID"
  data/1 -> Bus Creator/7  "Data"
  length/1 -> Data Type Conversion14/1
  Constant4/1 -> Data Type Conversion15/1
  CAN Unpack6/1 -> Data Type Conversion4/1
  CAN Unpack6/2 -> Data Type Conversion1/1
  CAN Unpack6/3 -> Data Type Conversion2/1
  Data Type Conversion4/1 -> Bus Creator1/1  "NH3_Store_g"
  Data Type Conversion1/1 -> Bus Creator1/2  "O2_frac_pct"
  Data Type Conversion2/1 -> Bus Creator1/3  "Regen_State"
  Add/1 -> Data Store Write/1
  Constant/1 -> Add/2
  Data Store Read/1 -> Add/1
  Data Type Conversion3/1 -> Bus Creator1/4  "Reserved_0700"
  CAN Unpack6/4 -> Data Type Conversion3/1

== system ECU1119_18b_st/SigIn/CAN2/Obj_Temp_Fb1/UNPACK ==
  ID : Inport
  data : Inport  Port=2
  length : Inport  Port=3
  timestamp : Inport  Port=4
  Action Port : ActionPort  ActionType=case
  Add : Sum
  Bus Creator : BusCreator  Inputs=7  OutDataTypeStr=Bus: CAN_MESSAGE_BUS  NonVirtualBus=on
  Bus Creator1 : BusCreator  Inputs=4
  CAN Unpack6 : canmsglib/CAN Unpack  CANdbFile=D:\VCU\VCU_Tractor_HaerBin\Tractor2\CANtest\ECU_CAN_st.dbc  MsgList=Obj_Temp_Fb1  MsgName=Obj_Temp_Fb1  MsgIDType=Standard (11-bit identifier)  MsgIdentifier=259  MsgLength=8  SignalInfo=DOC_In_Temp_C$0$16$1$2$1$0$1.000000e-01$0$0$1000$#DOC_Out_Temp_C$16$16$1$2$1$0$1.000000e-01$0$0$1000$#DPF_Out_Temp_C$32$16$1$2$1$0$1.000000e-01$0$0$1000$#SCR_In_Temp_C$48$16$1$2$1$0$1.000000e-01$0$0$1000$#  NSignals=4  IDPort=off  TimestampPort=off  ErrorPort=off  RemotePort=off  LengthPort=off  StatusPort=off  StartBits=str2num('[int32(0);int32(16);int32(32);int32(48)]')  SignalSizes=str2num('[int32(16);int32(16);int32(16);int32(16)]')  ByteOrders=str2num('[int32(1);int32(1);int32(1);int32(1)]')  DataTypes=str2num('[int32(2);int32(2);int32(2);int32(2)]')  MultiplexTypes=str2num('[int32(1);int32(1);int32(1);int32(1)]')  MultiplexValues=str2num('[double(0);double(0);double(0);double(0)]')  Factors=str2num('[double(1.000000e-01);double(1.000000e-01);double(1.000000e-01);double(1.000000e-01)]')  Offsets=str2num('[double(0);double(0);double(0);double(0)]')  Minimums=str2num('[double(0);double(0);double(0);double(0)]')  Maximums=str2num('[double(1000);double(1000);double(1000);double(1000)]')  ApplyMinMax=off
      settings: SourceProductName=Simulink Real-Time  SourceProductBaseCode=XP  DataFormat=CANdb specified signals
  Constant : Constant  OutDataTypeStr=uint8
  Constant1 : Constant  Value=0  OutDataTypeStr=uint8
  Constant4 : Constant  Value=0  OutDataTypeStr=uint8
  Constant5 : Constant  Value=0  OutDataTypeStr=uint8
  Data Store Read : DataStoreRead  DataStoreName=Cnt_TEMP1
  Data Store Write : DataStoreWrite  DataStoreName=Cnt_TEMP1
  Data Type Conversion{,14..15,17} (4 alike) : DataTypeConversion  OutDataTypeStr=uint8
  Data Type Conversion{1..4,19} (5 alike) : DataTypeConversion  OutDataTypeStr=double
  Data Type Conversion18 : DataTypeConversion  OutDataTypeStr=uint32
  Message : Outport
  wires:
  Bus Creator1/1 -> Message/1
  Data Type Conversion15/1 -> Bus Creator/3  "Remote"
  Data Type Conversion14/1 -> Bus Creator/2  "Length"
  Data Type Conversion/1 -> Bus Creator/1  "Extended"
  Bus Creator/1 -> CAN Unpack6/1  "CAN_Msg_In"
  Data Type Conversion17/1 -> Bus Creator/4  "Error"
  timestamp/1 -> Data Type Conversion19/1
  Data Type Conversion19/1 -> Bus Creator/6  "Timestamp"
  ID/1 -> Data Type Conversion18/1
  Constant5/1 -> Data Type Conversion17/1
  Constant1/1 -> Data Type Conversion/1
  Data Type Conversion18/1 -> Bus Creator/5  "ID"
  data/1 -> Bus Creator/7  "Data"
  length/1 -> Data Type Conversion14/1
  Constant4/1 -> Data Type Conversion15/1
  CAN Unpack6/1 -> Data Type Conversion3/1
  CAN Unpack6/2 -> Data Type Conversion2/1
  CAN Unpack6/3 -> Data Type Conversion1/1
  Data Type Conversion3/1 -> Bus Creator1/1  "DOC_In_Temp_C"
  Data Type Conversion2/1 -> Bus Creator1/2  "DOC_Out_Temp_C"
  Data Type Conversion1/1 -> Bus Creator1/3  "DPF_Out_Temp_C"
  Add/1 -> Data Store Write/1
  Constant/1 -> Add/2
  Data Store Read/1 -> Add/1
  Data Type Conversion4/1 -> Bus Creator1/4  "SCR_In_Temp_C"
  CAN Unpack6/4 -> Data Type Conversion4/1

== system ECU1119_18b_st/SigIn/CAN2/Obj_Temp_Fb2/UNPACK ==
  ID : Inport
  data : Inport  Port=2
  length : Inport  Port=3
  timestamp : Inport  Port=4
  Action Port : ActionPort  ActionType=case
  Add : Sum
  Bus Creator : BusCreator  Inputs=7  OutDataTypeStr=Bus: CAN_MESSAGE_BUS  NonVirtualBus=on
  Bus Creator1 : BusCreator  Inputs=3
  CAN Unpack6 : canmsglib/CAN Unpack  CANdbFile=D:\VCU\VCU_Tractor_HaerBin\Tractor2\CANtest\ECU_CAN_st.dbc  MsgList=Obj_Temp_Fb2  MsgName=Obj_Temp_Fb2  MsgIDType=Standard (11-bit identifier)  MsgIdentifier=260  MsgLength=8  SignalInfo=ExhMassFlow_kgph$16$16$1$2$1$0$1.000000e-01$0$0$2000$#Reserved_0500$32$32$1$2$1$0$1$0$0$4294967295$#SCR_Out_Temp_C$0$16$1$2$1$0$1.000000e-01$0$0$1000$#  NSignals=3  IDPort=off  TimestampPort=off  ErrorPort=off  RemotePort=off  LengthPort=off  StatusPort=off  StartBits=str2num('[int32(16);int32(32);int32(0)]')  SignalSizes=str2num('[int32(16);int32(32);int32(16)]')  ByteOrders=str2num('[int32(1);int32(1);int32(1)]')  DataTypes=str2num('[int32(2);int32(2);int32(2)]')  MultiplexTypes=str2num('[int32(1);int32(1);int32(1)]')  MultiplexValues=str2num('[double(0);double(0);double(0)]')  Factors=str2num('[double(1.000000e-01);double(1);double(1.000000e-01)]')  Offsets=str2num('[double(0);double(0);double(0)]')  Minimums=str2num('[double(0);double(0);double(0)]')  Maximums=str2num('[double(2000);double(4294967295);double(1000)]')  ApplyMinMax=off
      settings: SourceProductName=Simulink Real-Time  SourceProductBaseCode=XP  DataFormat=CANdb specified signals
  Constant : Constant  OutDataTypeStr=uint8
  Constant1 : Constant  Value=0  OutDataTypeStr=uint8
  Constant4 : Constant  Value=0  OutDataTypeStr=uint8
  Constant5 : Constant  Value=0  OutDataTypeStr=uint8
  Data Store Read : DataStoreRead  DataStoreName=Cnt_TEMP2
  Data Store Write : DataStoreWrite  DataStoreName=Cnt_TEMP2
  Data Type Conversion{,14..15,17} (4 alike) : DataTypeConversion  OutDataTypeStr=uint8
  Data Type Conversion{1..2,4,19} (4 alike) : DataTypeConversion  OutDataTypeStr=double
  Data Type Conversion18 : DataTypeConversion  OutDataTypeStr=uint32
  Message : Outport
  wires:
  Data Store Read/1 -> Add/1
  Constant/1 -> Add/2
  Add/1 -> Data Store Write/1
  Data Type Conversion2/1 -> Bus Creator1/3  "SCR_Out_Temp_C"
  Data Type Conversion1/1 -> Bus Creator1/2  "Reserved_0500"
  Data Type Conversion4/1 -> Bus Creator1/1  "ExhMassFlow_kgph"
  CAN Unpack6/3 -> Data Type Conversion2/1
  CAN Unpack6/2 -> Data Type Conversion1/1
  CAN Unpack6/1 -> Data Type Conversion4/1
  Constant4/1 -> Data Type Conversion15/1
  length/1 -> Data Type Conversion14/1
  data/1 -> Bus Creator/7  "Data"
  Data Type Conversion18/1 -> Bus Creator/5  "ID"
  Constant1/1 -> Data Type Conversion/1
  Constant5/1 -> Data Type Conversion17/1
  ID/1 -> Data Type Conversion18/1
  Data Type Conversion19/1 -> Bus Creator/6  "Timestamp"
  timestamp/1 -> Data Type Conversion19/1
  Data Type Conversion17/1 -> Bus Creator/4  "Error"
  Bus Creator/1 -> CAN Unpack6/1  "CAN_Msg_In"
  Data Type Conversion/1 -> Bus Creator/1  "Extended"
  Data Type Conversion14/1 -> Bus Creator/2  "Length"
  Data Type Conversion15/1 -> Bus Creator/3  "Remote"
  Bus Creator1/1 -> Message/1

== system ECU1119_18b_st/SigIn/PWM/PWM_PTS1/Subsystem ==
  In1 : Inport
  Add2 : Sum  AccumDataTypeStr=single
  Constant : Constant  OutDataTypeStr=uint8
  Constant1 : Constant  Value=0  OutDataTypeStr=single
  Data Store Read3 : DataStoreRead  DataStoreName=pts1_pwm_cnt
  Data Store Write : DataStoreWrite  DataStoreName=pts1_pwm_cnt
  Saturation : Saturate  UpperLimit=100  LowerLimit=0
  Switch : Switch  Criteria=u2 > Threshold  Threshold=100
  Out1 : Outport  VectorParamsAs1DForOutWhenUnconnected=on
  wires:
  Saturation/1 -> Data Store Write/1
  Add2/1 -> Switch/2, Saturation/1
  Data Store Read3/1 -> Add2/2
  Constant1/1 -> Switch/1
  Switch/1 -> Out1/1
  Constant/1 -> Add2/1
  In1/1 -> Switch/3

== system ECU1119_18b_st/SigIn/PWM/PWM_PTS1/Subsystem_capture ==
  In1 : Inport
  function : TriggerPort  TriggerType=function-call  VariantControl=Variant
  Constant : Constant  Value=0  OutDataTypeStr=uint8
  Counter Limited : simulink/Sources/Counter Limited  uplimit=7  tsamp=-1
  Data Store Write : DataStoreWrite  DataStoreName=pts1_pwm_cnt
  Data Store Write3 : DataStoreWrite  DataStoreName=pwm3_cnt
  Terminator : Terminator
  eTimer_Arm_Capture : mbd_mpc574x_ec_toolbox/Motor Control Blocks/eTIMER Blocks/eTimer_Arm_Capture  etimerModule=1  etimerChannel=2  etimerArmAction=Stop
      settings: SourceProductName=NXP Model-Based Design Toolbox for MPC57xx MCUs
  eTimer_Capture : mbd_mpc574x_ec_toolbox/Motor Control Blocks/eTIMER Blocks/eTimer_Capture  etimerModule=1  etimerChannel=2
      settings: SourceProductName=NXP Model-Based Design Toolbox for MPC57xx MCUs
  Out1 : Outport  OutDataTypeStr=uint16
  Out2 : Outport  Port=2  OutDataTypeStr=uint16
  Out3 : Outport  Port=3  OutDataTypeStr=uint16
  Out4 : Outport  Port=4  OutDataTypeStr=uint16
  wires:
  eTimer_Capture/1 -> Out1/1
  eTimer_Capture/4 -> Out4/1
  eTimer_Capture/3 -> Out3/1
  eTimer_Capture/2 -> Out2/1
  In1/1 -> Terminator/1
  Constant/1 -> Data Store Write/1
  Counter Limited/1 -> Data Store Write3/1

== system ECU1119_18b_st/SigIn/PWM/PWM_PTS2/Subsystem ==
  In1 : Inport
  Add2 : Sum  AccumDataTypeStr=single
  Constant : Constant  OutDataTypeStr=uint8
  Constant1 : Constant  Value=0  OutDataTypeStr=single
  Data Store Read3 : DataStoreRead  DataStoreName=pts2_pwm_cnt
  Data Store Write : DataStoreWrite  DataStoreName=pts2_pwm_cnt
  Saturation : Saturate  UpperLimit=100  LowerLimit=0
  Switch : Switch  Criteria=u2 > Threshold  Threshold=100
  Out1 : Outport  VectorParamsAs1DForOutWhenUnconnected=on
  wires:
  In1/1 -> Switch/3
  Constant/1 -> Add2/1
  Switch/1 -> Out1/1
  Constant1/1 -> Switch/1
  Data Store Read3/1 -> Add2/2
  Add2/1 -> Saturation/1, Switch/2
  Saturation/1 -> Data Store Write/1

== system ECU1119_18b_st/SigIn/PWM/PWM_PTS2/Subsystem_capture ==
  In1 : Inport
  function : TriggerPort  TriggerType=function-call  VariantControl=Variant
  Constant : Constant  Value=0  OutDataTypeStr=uint8
  Counter Limited : simulink/Sources/Counter Limited  uplimit=255  tsamp=-1
  Data Store Write : DataStoreWrite  DataStoreName=pts2_pwm_cnt
  Data Store Write2 : DataStoreWrite  DataStoreName=pwm2_cnt
  Terminator : Terminator
  eTimer_Arm_Capture : mbd_mpc574x_ec_toolbox/Motor Control Blocks/eTIMER Blocks/eTimer_Arm_Capture  etimerModule=1  etimerChannel=3  etimerArmAction=Stop
      settings: SourceProductName=NXP Model-Based Design Toolbox for MPC57xx MCUs
  eTimer_Capture : mbd_mpc574x_ec_toolbox/Motor Control Blocks/eTIMER Blocks/eTimer_Capture  etimerModule=1  etimerChannel=3
      settings: SourceProductName=NXP Model-Based Design Toolbox for MPC57xx MCUs
  Out1 : Outport  OutDataTypeStr=uint16
  Out2 : Outport  Port=2  OutDataTypeStr=uint16
  Out3 : Outport  Port=3  OutDataTypeStr=uint16
  Out4 : Outport  Port=4  OutDataTypeStr=uint16
  wires:
  Constant/1 -> Data Store Write/1
  In1/1 -> Terminator/1
  eTimer_Capture/2 -> Out2/1
  eTimer_Capture/3 -> Out3/1
  eTimer_Capture/4 -> Out4/1
  eTimer_Capture/1 -> Out1/1
  Counter Limited/1 -> Data Store Write2/1

== system ECU1119_18b_st/SigIn/PWM/PWM_PTS3/Subsystem ==
  In1 : Inport
  Add2 : Sum  AccumDataTypeStr=single
  Constant : Constant  OutDataTypeStr=uint8
  Constant1 : Constant  Value=0  OutDataTypeStr=single
  Data Store Read3 : DataStoreRead  DataStoreName=pts3_pwm_cnt
  Data Store Write : DataStoreWrite  DataStoreName=pts3_pwm_cnt
  Saturation : Saturate  UpperLimit=100  LowerLimit=0
  Switch : Switch  Criteria=u2 > Threshold  Threshold=100
  Out1 : Outport  VectorParamsAs1DForOutWhenUnconnected=on
  wires:
  Saturation/1 -> Data Store Write/1
  Add2/1 -> Switch/2, Saturation/1
  Data Store Read3/1 -> Add2/2
  Constant1/1 -> Switch/1
  Switch/1 -> Out1/1
  Constant/1 -> Add2/1
  In1/1 -> Switch/3
